simulink model "LabB_PIDOverRobot"  (R2017a)
settings: Solver=FixedStepDiscrete  StartTime=0.0  StopTime=inf  FixedStep=fSamplingPeriod  RelTol=1e-3  EnableMultiTasking=on
values from neighbouring files (symbols this model uses):
  fGyroBias = 125.292978208    [GyroBias.mat]    (also in LabB_TuneTheGyro_SaveParameters.m = mean(afGyroBias.signals.values))
  fGyroConversionFactor = -1/131    (= -0.00763358778626)    [LabB_PIDOverRobot_Parameters.m]    (also in LoadRobotParameters.m = 0.00762939453125)
  fSamplingPeriod = 0.01    [LabB_CheckCommunications_Parameters.m]    (also in LabB_ControllerOverSimulator_Discrete_Parameters.m = 0.005; LabB_ObserverOverSimulator_Discrete_Parameters.m = 0.005; LabB_PIDOverRobot_Parameters.m = 0.005; LabB_TuneTheGyro_SaveParameters.m)
  fWheelRadius = 0.0216    [LabB_PIDOverRobot_Parameters.m]    (also in LoadRobotParameters.m)
  iNumberOfEncoderSteps = 720    [LabB_PIDOverRobot_Parameters.m]    (also in LoadRobotParameters.m)
  kD = -0.1    [LabB_ObserverOverSimulator_Continuous_Parameters.m]    (also in LabB_ObserverOverSimulator_Discrete_Parameters.m; LabB_PIDOverRobot_Parameters.m = -0.1302; matlab.mat = 4.36540372554)
  kI = -260    [LabB_ObserverOverSimulator_Continuous_Parameters.m]    (also in LabB_ObserverOverSimulator_Discrete_Parameters.m; LabB_PIDOverRobot_Parameters.m = -390.4363; matlab.mat = -279.677756448)
  kP = -46.6    [LabB_ObserverOverSimulator_Continuous_Parameters.m]    (also in LabB_ObserverOverSimulator_Discrete_Parameters.m; LabB_PIDOverRobot_Parameters.m = -69.6802; matlab.mat = -28.3577737752)
undefined symbols (not defined in the file or in its folder): DiscIntNeverNeededParam
libraries: simulink x15, MinSegLibrary_M2V3 x2, arduinolib x1
settings Model: FPTRunName=FPA_Reference  SimulationMode=external  ExtModeTrigDuration=2  Creator=Alec  LastModifiedBy=damiano
settings DataIOCC: SaveFormat=Array  SaveOutput=off  SignalLogging=off  DSMLogging=off  SaveTime=off
settings OptimizationCC: PassReuseOutputArgsAs=Individual arguments  ExpressionDepthLimit=2147483647  MaxStackSize=64
settings DebuggingCC: UnderspecifiedInitializationDetection=Classic  MergeDetectMultiDrivingBlocksExec=none  ParameterTunabilityLossMsg=error  StateNameClashWarn=warning  SFUnexpectedBacktrackingDiag=warning  SFNoUnconditionalDefaultTransitionDiag=warning  SFExecutionAtInitializationDiag=none
settings HardwareCC: ProdBitPerInt=16  ProdBitPerPointer=16  ProdBitPerSizeT=16  ProdBitPerPtrDiffT=16  ProdLargestAtomicFloat=None  ProdWordSize=8  ProdHWDeviceType=Atmel->AVR
settings ModelReferenceCC: PropagateSignalLabelsOutOfModel=off
settings SFSimCC: MATLABDynamicMemAlloc=off
settings RTWCC: SystemTargetFile=ert.tlc  HardwareBoard=Arduino Mega 2560  TLCOptions=-aInlineSetEventsForThisBaseRateFcn=TLC_FALSE -aSuppressMultiTaskScheduler=TLC_FALSE -aRateBasedStepFcn=1  TemplateMakefile=ert_default_tmf  Description=Embedded Coder  GenerateReport=on  RTWVerbose=off  Toolchain=Arduino AVR  BuildConfiguration=Faster Runs  IncludeHyperlinkInReport=on  LaunchReport=on  GenerateTraceInfo=on  GenerateTraceReport=on  GenerateTraceReportSl=on  GenerateTraceReportSf=on  GenerateTraceReportEml=on
settings CodeAppCC: ForceParamTrailComments=on  IgnoreCustomStorageClasses=off  OperatorAnnotations=on  SimulinkDataObjDesc=on  SFDataObjDesc=on  MATLABFcnDesc=on  CustomSymbolStrType=$N$R$M  InsertBlockDesc=on  MATLABSourceComments=on  InternalIdentifier=Classic
settings ERTTargetCC: SupportContinuousTime=on  SupportVariableSizeSignals=on
settings ConfigComp: CovMetricSettings=dw  CovHtmlReporting=on  CovSaveCumulativeToWorkspaceVar=on  CovSaveSingleToWorkspaceVar=on  CovExternalEMLEnable=off

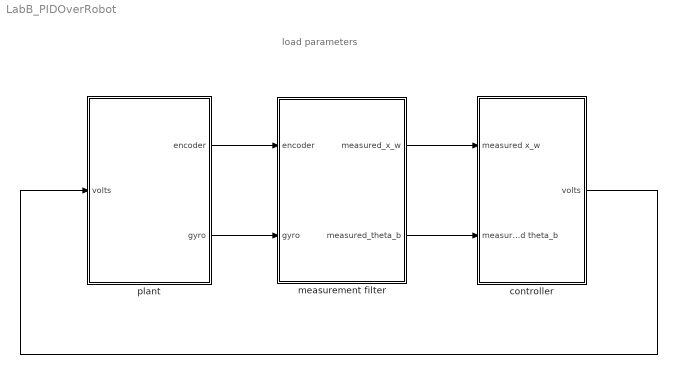
== system LabB_PIDOverRobot ==
  note: load parameters
  controller : Subsystem
  measurement filter : Subsystem
  plant : Subsystem
  wires:
  controller/1(volts) -> plant/1(volts)
  plant/2(gyro) -> measurement filter/2(gyro)
  measurement filter/2(measured_theta_b) -> controller/2("measured theta_b ")
  measurement filter/1(measured_x_w) -> controller/1(measured x_w)
  plant/1(encoder) -> measurement filter/1(encoder)

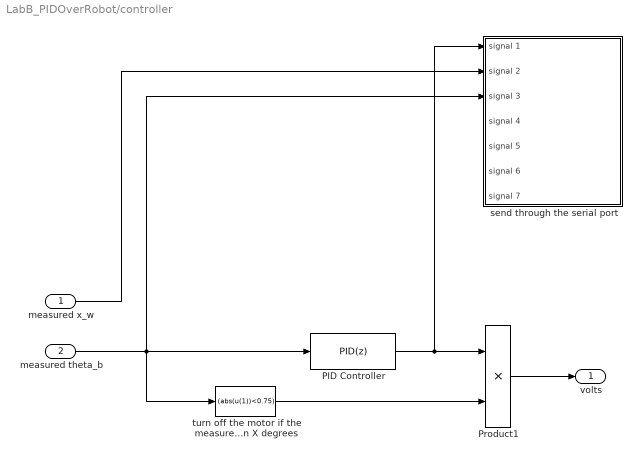
== system LabB_PIDOverRobot/controller ==
  measured x_w : Inport
  "measured theta_b " : Inport  Port=2
  PID Controller : simulink/Continuous/PID Controller  Controller=PID  TimeDomain=Discrete-time  SampleTime=fSamplingPeriod  IntegratorMethod=Forward Euler  FilterMethod=Forward Euler  Form=Parallel  UseFilter=on  ControllerParametersSource=internal  P=-kP  I=-kI  D=-kD  N=100  InitialConditionSource=internal  InitialConditionForIntegrator=0  InitialConditionForFilter=0  ExternalReset=none  LimitOutput=on  UpperSaturationLimit=6  LowerSaturationLimit=-6  LinearizeAsGain=on  AntiWindupMode=back-calculation  Kb=1  TrackingMode=off  Kt=1  PParamMin=[]  PParamMax=[]  IParamMin=[]  IParamMax=[]  DParamMin=[]  DParamMax=[]  NParamMin=[]  NParamMax=[]  KbParamMin=[]  KbParamMax=[]  KtParamMin=[]  KtParamMax=[]  POutMin=[]  POutMax=[]  IOutMin=[]  IOutMax=[]  DOutMin=[]  DOutMax=[]  NOutMin=[]  NOutMax=[]  KbOutMin=[]  KbOutMax=[]  KtOutMin=[]  KtOutMax=[]  IntegratorOutMin=[]  IntegratorOutMax=[]  FilterOutMin=[]  FilterOutMax=[]  SumOutMin=[]  SumOutMax=[]  SumI1OutMin=[]  SumI1OutMax=[]  SumI2OutMin=[]  SumI2OutMax=[]  SumI3OutMin=[]  SumI3OutMax=[]  SumDOutMin=[]  SumDOutMax=[]  SaturationOutMin=[]  SaturationOutMax=[]  IntegratorContinuousStateAttributes=''  IntegratorStateMustResolveToSignalObject=off  IntegratorRTWStateStorageClass=Auto  FilterContinuousStateAttributes=''  FilterStateMustResolveToSignalObject=off  FilterRTWStateStorageClass=Auto  DifferentiatorICPrevScaledInput=0  DifferentiatorOutMin=[]  DifferentiatorOutMax=[]  InitialConditionSetting=State (most efficient)
  Product1 : Product  RndMeth=Zero
  send through the serial port : Subsystem
  turn off the motor if the measured angle is greater than X degrees : Fcn  Expr=(abs(u(1))<0.75)
  volts : Outport
  wires:
  "measured theta_b "/1 -> send through the serial port/3(signal 3), turn off the motor if the measured angle is greater than X degrees/1, PID Controller/1
  Product1/1 -> volts/1
  turn off the motor if the measured angle is greater than X degrees/1 -> Product1/2
  PID Controller/1 -> send through the serial port/1(signal 1), Product1/1
  measured x_w/1 -> send through the serial port/2(signal 2)

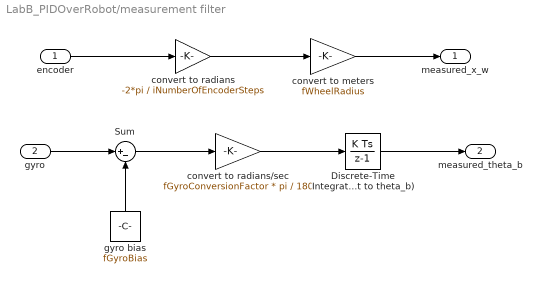
== system LabB_PIDOverRobot/measurement filter ==
  encoder : Inport
  gyro : Inport  Port=2
  Discrete-Time Integrator (convert from theta_b_dot to theta_b) : DiscreteIntegrator  SampleTime=fSamplingPeriod  OutDataTypeStr=Inherit: Inherit via back propagation  ICPrevOutput=DiscIntNeverNeededParam  ICPrevScaledInput=DiscIntNeverNeededParam
  Sum : Sum  Inputs=|+-
  convert to radians/sec : Gain  Gain=fGyroConversionFactor * pi / 180  OutDataTypeStr=Inherit: Same as input
  convert to radians : Gain  Gain=-2*pi / iNumberOfEncoderSteps  OutDataTypeStr=Inherit: Same as input
  convert to meters : Gain  Gain=fWheelRadius  OutDataTypeStr=Inherit: Same as input
  gyro bias : Constant  Value=fGyroBias  OutDataTypeStr=single
  measured_x_w : Outport
  measured_theta_b : Outport  Port=2
  wires:
  convert to radians/sec/1 -> Discrete-Time Integrator (convert from theta_b_dot to theta_b)/1
  gyro/1 -> Sum/1
  Sum/1 -> convert to radians/sec/1
  convert to radians/1 -> convert to meters/1
  encoder/1 -> convert to radians/1
  Discrete-Time Integrator (convert from theta_b_dot to theta_b)/1 -> measured_theta_b/1
  gyro bias/1 -> Sum/2
  convert to meters/1 -> measured_x_w/1

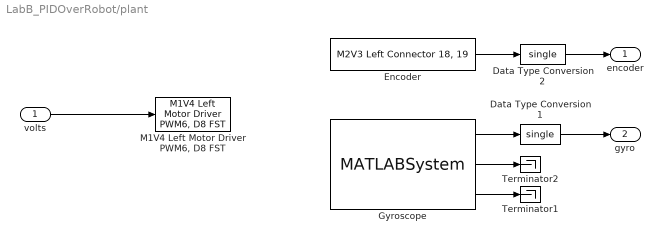
== system LabB_PIDOverRobot/plant ==
  volts : Inport
  Data Type Conversion1 : DataTypeConversion  OutDataTypeStr=single
  Data Type Conversion2 : DataTypeConversion  OutDataTypeStr=single
  Encoder : MinSegLibrary_M2V3/M2V3 Left Connector 18, 19  Encoder=1  PinA=19  PinB=18  PWMFSelect=1  PWMTimer=3
      settings: SourceProductName=Rensselaer Arduino Support Package
  Gyroscope : MATLABSystem  System=soMPU6050Gyro  DLPFmode=0
      mask Type: soMPU6050Gyro
      mask Display:
      | disp('soMPU6050Gyro');
      | port_label('output',1,'xvel');
      | port_label('output',2,'yvel');
      | port_label('output',3,'zvel');
  "M1V4 Left Motor Driver PWM6, D8 FST" : MinSegLibrary_M2V3/M1V4 Left Motor Driver PWM6, D8 FST  Vsupply=9
      settings: SourceProductName=Rensselaer Arduino Support Package
  Terminator1 : Terminator
  Terminator2 : Terminator
  encoder : Outport
  gyro : Outport  Port=2
  wires:
  Gyroscope/1 -> Data Type Conversion1/1
  Data Type Conversion1/1 -> gyro/1
  Encoder/1 -> Data Type Conversion2/1
  Data Type Conversion2/1 -> encoder/1
  Gyroscope/3 -> Terminator1/1
  Gyroscope/2 -> Terminator2/1
  volts/1 -> "M1V4 Left Motor Driver PWM6, D8 FST"/1

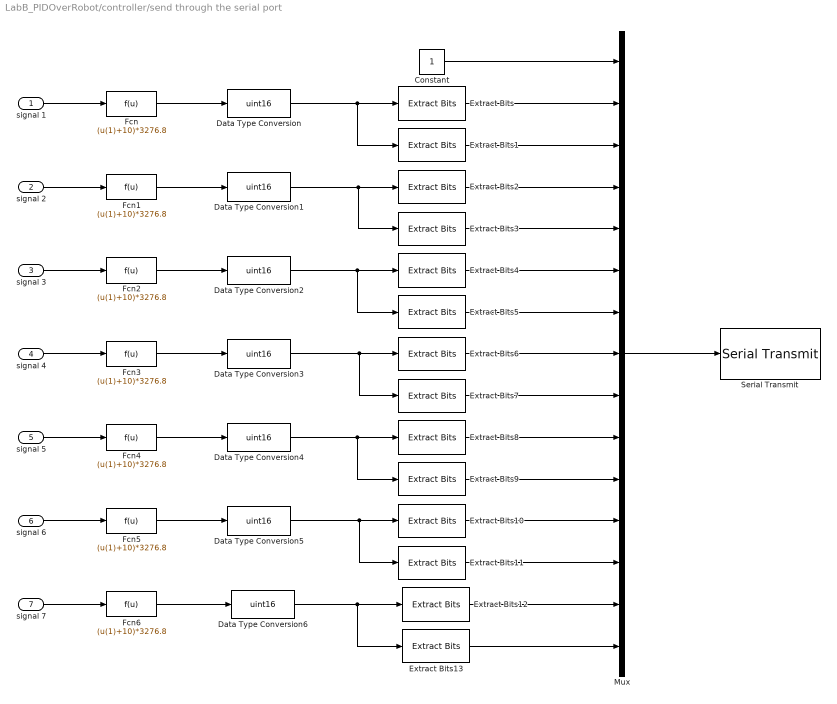
== system LabB_PIDOverRobot/controller/send through the serial port ==
  signal 1 : Inport
  signal 2 : Inport  Port=2
  signal 3 : Inport  Port=3
  signal 4 : Inport  Port=4
  signal 5 : Inport  Port=5
  signal 6 : Inport  Port=6
  signal 7 : Inport  Port=7
  Constant : Constant  OutDataTypeStr=uint8
  Data Type Conversion{,1..6} (7 alike) : DataTypeConversion  OutDataTypeStr=uint16
  Extract Bits{,2,4,6,8,10,12} (7 alike) : simulink/Logic and Bit Operations/Extract Bits  bitsToExtract=Upper half  numBits=8  bitIdxRange=[0 7]  outScalingMode=Treat bit field as an integer
      settings: SourceProductName=Simulink
  Extract Bits{1,3,5,7,9,11,13} (7 alike) : simulink/Logic and Bit Operations/Extract Bits  bitsToExtract=Lower half  numBits=8  bitIdxRange=[0 7]  outScalingMode=Treat bit field as an integer
      settings: SourceProductName=Simulink
  Fcn{,1..6} (7 alike) : Fcn  Expr=(u(1)+10)*3276.8
  Mux : Mux  Inputs=15
  Serial Transmit : arduinolib/Serial Transmit  portNumber=0  sendmode=write  sendformat=Decimal  floatprecision=2  blockPlatform=arduino
      settings: SourceProductName=Simulink Support Package for Arduino Hardware
  wires:
  Data Type Conversion/1 -> Extract Bits1/1, Extract Bits/1
  Extract Bits/1 -> Mux/2
  Fcn1/1 -> Data Type Conversion1/1
  Fcn/1 -> Data Type Conversion/1
  Extract Bits2/1 -> Mux/4
  Constant/1 -> Mux/1
  Data Type Conversion1/1 -> Extract Bits2/1, Extract Bits3/1
  Extract Bits1/1 -> Mux/3
  Mux/1 -> Serial Transmit/1
  Extract Bits3/1 -> Mux/5
  Data Type Conversion3/1 -> Extract Bits6/1, Extract Bits7/1
  Extract Bits4/1 -> Mux/6
  Data Type Conversion2/1 -> Extract Bits5/1, Extract Bits4/1
  Extract Bits5/1 -> Mux/7
  Extract Bits6/1 -> Mux/8
  Fcn3/1 -> Data Type Conversion3/1
  Extract Bits7/1 -> Mux/9
  Fcn2/1 -> Data Type Conversion2/1
  Data Type Conversion4/1 -> Extract Bits9/1, Extract Bits8/1
  Fcn5/1 -> Data Type Conversion5/1
  Extract Bits8/1 -> Mux/10
  Extract Bits9/1 -> Mux/11
  Data Type Conversion5/1 -> Extract Bits10/1, Extract Bits11/1
  Extract Bits11/1 -> Mux/13
  Extract Bits10/1 -> Mux/12
  Fcn4/1 -> Data Type Conversion4/1
  signal 2/1 -> Fcn1/1
  signal 7/1 -> Fcn6/1
  signal 6/1 -> Fcn5/1
  signal 3/1 -> Fcn2/1
  signal 1/1 -> Fcn/1
  signal 4/1 -> Fcn3/1
  signal 5/1 -> Fcn4/1
  Extract Bits13/1 -> Mux/15
  Extract Bits12/1 -> Mux/14
  Fcn6/1 -> Data Type Conversion6/1
  Data Type Conversion6/1 -> Extract Bits12/1, Extract Bits13/1
